simulink model "gtm_design"  (R2020b)
settings: Solver=ode3  StartTime=0.0  StopTime=20  FixedStep=Timestep  MaxStep=0.1  MinStep=0.005  RelTol=1e-5
StopFcn:
  | MWSout=grabmws(bdroot);
  | MWSout.lastrun=datestr(now);
values from neighbouring files (symbols this model uses):
  AILL = simout.surf.AILL.Data    [plot_result.m]
  AILR = simout.surf.AILR.Data    [plot_result.m]
  ELLIB = simout.surf.ELLIB.Data    [plot_result.m]
  ELLOB = simout.surf.ELLOB.Data    [plot_result.m]
  ELRIB = simout.surf.ELRIB.Data    [plot_result.m]
  ELROB = simout.surf.ELROB.Data    [plot_result.m]
  RUDL = simout.surf.RUDL.Data    [plot_result.m]
  RUDU = simout.surf.RUDU.Data    [plot_result.m]
  THROTL = simout.surf.THROTL.Data    [plot_result.m]
  THROTR = simout.surf.THROTR.Data    [plot_result.m]
undefined symbols (not defined in the file or in its folder): Aero, aftfuel, aftfuel_pos, AILLC, AILRC, alpha_deg, altitude_ft, Ax_g, Ay_g, Az_g, b, beta_deg, bias, BRAKEC, Cbar, cg_pos0, cg_shift_gear, DamageCase, DamageModels, DamageOnsetTime, ELLIBC, ELLOBC, ELRIBC, ELROBC, engl_ang, engl_pos, engr_ang, engr_pos, FLAPLIB, FLAPLIC, FLAPLOB, FLAPLOC, FLAPRIB, FLAPRIC, FLAPROB, FLAPROC, FuelUsed_Init, fwdfuel, fwdfuel_pos, GEAR, GEARC, Inertia0, Inertia_shift_gear, Ixx_model, Iyy_model, Izz_model, KTAS, LandingGear, LengON, LinearizeModeOn, NAV_altitude_m, NAV_latitude_deg, NAV_longitude_deg, NAV_Ve_mps, NAV_Vn_mps, NAV_Vu_mps, Newton, p_deg, phi_deg, POS_hi ... (+40)
libraries: simulink_need_slupdate x40, simulink x4, simulink_extras x3, UserContent_lib x1
(part 4 of 6)

== system gtm_design/GTM_T2/Actuators/Acutator Dynamics/RudderLServo ==
  In : Inport
  Constant : Constant  Value=Bias
  Gain : Gain  Gain=2*pi*freq  SaturateOnIntegerOverflow=on  OutDataTypeStr=Inherit: Same as input  ParamDataTypeStr=Inherit: Same as input
  Integrator : Integrator  InitialConditionSource=external  LimitOutput=on  UpperSaturationLimit=POS_hi  LowerSaturationLimit=POS_lo  IgnoreLimit=on
  Rate Limiter : Saturate  UpperLimit=RL  LowerLimit=-RL
  Sum : Sum  Inputs=-+|  InputSameDT=on  SaturateOnIntegerOverflow=on  OutDataTypeStr=Inherit: Same as first input
  Sum1 : Sum  Inputs=++|  InputSameDT=on  SaturateOnIntegerOverflow=on  OutDataTypeStr=Inherit: Same as first input
  Out : Outport  PortDimensions=1  VectorParamsAs1DForOutWhenUnconnected=off
  wires:
  Constant/1 -> Sum1/1
  Sum1/1 -> Integrator/2, Sum/2
  In/1 -> Sum1/2
  Rate Limiter/1 -> Integrator/1  "Ydot_lim"
  Integrator/1 -> Out/1, Sum/1  "Y"
  Sum/1 -> Gain/1  "Error"
  Gain/1 -> Rate Limiter/1  "Ydot"

== system gtm_design/GTM_T2/Actuators/Acutator Dynamics/RudderUServo ==
  In : Inport
  Constant : Constant  Value=Bias
  Gain : Gain  Gain=2*pi*freq  SaturateOnIntegerOverflow=on  OutDataTypeStr=Inherit: Same as input  ParamDataTypeStr=Inherit: Same as input
  Integrator : Integrator  InitialConditionSource=external  LimitOutput=on  UpperSaturationLimit=POS_hi  LowerSaturationLimit=POS_lo  IgnoreLimit=on
  Rate Limiter : Saturate  UpperLimit=RL  LowerLimit=-RL
  Sum : Sum  Inputs=-+|  InputSameDT=on  SaturateOnIntegerOverflow=on  OutDataTypeStr=Inherit: Same as first input
  Sum1 : Sum  Inputs=++|  InputSameDT=on  SaturateOnIntegerOverflow=on  OutDataTypeStr=Inherit: Same as first input
  Out : Outport  PortDimensions=1  VectorParamsAs1DForOutWhenUnconnected=off
  wires:
  Constant/1 -> Sum1/1
  Sum1/1 -> Integrator/2, Sum/2
  In/1 -> Sum1/2
  Rate Limiter/1 -> Integrator/1  "Ydot_lim"
  Integrator/1 -> Out/1, Sum/1  "Y"
  Sum/1 -> Gain/1  "Error"
  Gain/1 -> Rate Limiter/1  "Ydot"

== system gtm_design/GTM_T2/Actuators/Acutator Dynamics/SteeringServo ==
  In : Inport
  Constant : Constant  Value=Bias
  Gain : Gain  Gain=2*pi*freq  SaturateOnIntegerOverflow=on  OutDataTypeStr=Inherit: Same as input  ParamDataTypeStr=Inherit: Same as input
  Integrator : Integrator  InitialConditionSource=external  LimitOutput=on  UpperSaturationLimit=POS_hi  LowerSaturationLimit=POS_lo  IgnoreLimit=on
  Rate Limiter : Saturate  UpperLimit=RL  LowerLimit=-RL
  Sum : Sum  Inputs=-+|  InputSameDT=on  SaturateOnIntegerOverflow=on  OutDataTypeStr=Inherit: Same as first input
  Sum1 : Sum  Inputs=++|  InputSameDT=on  SaturateOnIntegerOverflow=on  OutDataTypeStr=Inherit: Same as first input
  Out : Outport  PortDimensions=1  VectorParamsAs1DForOutWhenUnconnected=off
  wires:
  Constant/1 -> Sum1/1
  Sum1/1 -> Integrator/2, Sum/2
  In/1 -> Sum1/2
  Rate Limiter/1 -> Integrator/1  "Ydot_lim"
  Integrator/1 -> Out/1, Sum/1  "Y"
  Sum/1 -> Gain/1  "Error"
  Gain/1 -> Rate Limiter/1  "Ydot"

== system gtm_design/GTM_T2/Actuators/DeadBand/Deadband ==
  In : Inport
  Bus Assignment : BusAssignment  AssignedSignals=ELLOB,ELLIB,ELROB,ELRIB,AILL,AILR,RUDU,RUDL,FLAPLIB,FLAPLOB,FLAPRIB,FLAPROB
  Bus Selector : BusSelector  OutputSignals=ELLOB,ELLIB,ELROB,ELRIB,AILL,AILR,RUDU,RUDL,FLAPLIB,FLAPLOB,FLAPRIB,FLAPROB
  Dead Zone : DeadZone  LowerValue=-0.3  UpperValue=0.3  SaturateOnIntegerOverflow=on
  Dead Zone1 : DeadZone  LowerValue=-0.6  UpperValue=0.6  SaturateOnIntegerOverflow=on
  Dead Zone{6,12..15} (5 alike) : DeadZone  LowerValue=-0.4  UpperValue=0.4  SaturateOnIntegerOverflow=on
  Dead Zone2 : DeadZone  LowerValue=-0.3  UpperValue=0.3  SaturateOnIntegerOverflow=on
  Dead Zone3 : DeadZone  LowerValue=-0.6  UpperValue=0.6  SaturateOnIntegerOverflow=on
  Dead Zone4 : DeadZone  LowerValue=-0.25  UpperValue=0.25  SaturateOnIntegerOverflow=on
  Dead Zone5 : DeadZone  LowerValue=-0.25  UpperValue=0.25  SaturateOnIntegerOverflow=on
  Dead Zone7 : DeadZone  LowerValue=-0.3  UpperValue=0.3  SaturateOnIntegerOverflow=on
  Out : Outport  VectorParamsAs1DForOutWhenUnconnected=off
  wires:
  Bus Selector/1 -> Dead Zone/1  "<ELLOB>"
  Bus Selector/2 -> Dead Zone1/1  "<ELLIB>"
  Bus Selector/3 -> Dead Zone2/1  "<ELROB>"
  Bus Selector/4 -> Dead Zone3/1  "<ELRIB>"
  Bus Selector/5 -> Dead Zone4/1  "<AILL>"
  Bus Selector/6 -> Dead Zone5/1  "<AILR>"
  Bus Selector/7 -> Dead Zone6/1  "<RUDU>"
  Bus Selector/8 -> Dead Zone7/1  "<RUDL>"
  Bus Selector/9 -> Dead Zone12/1  "<FLAPLIB>"
  Bus Selector/10 -> Dead Zone13/1  "<FLAPLOB>"
  Bus Selector/11 -> Dead Zone14/1  "<FLAPRIB>"
  Bus Selector/12 -> Dead Zone15/1  "<FLAPROB>"
  Dead Zone/1 -> Bus Assignment/2
  Dead Zone1/1 -> Bus Assignment/3
  Dead Zone2/1 -> Bus Assignment/4
  Dead Zone3/1 -> Bus Assignment/5
  Dead Zone4/1 -> Bus Assignment/6
  Dead Zone5/1 -> Bus Assignment/7
  Dead Zone6/1 -> Bus Assignment/8
  Dead Zone7/1 -> Bus Assignment/9
  Dead Zone12/1 -> Bus Assignment/10
  Dead Zone13/1 -> Bus Assignment/11
  Dead Zone14/1 -> Bus Assignment/12
  Dead Zone15/1 -> Bus Assignment/13
  In/1 -> Bus Assignment/1, Bus Selector/1
  Bus Assignment/1 -> Out/1

== system gtm_design/GTM_T2/Actuators/InputModification for Trimming/Invalid, Error Out ==
  Action Port : ActionPort  ActionPortLabel=default:
  Constant1 : Constant  Value=zeros(22,1)
  Constant2 : Constant  Value=0
  InvalidMode : Assertion  AssertionFailFcn="warndlg('Invalid settings for TrimMode and LinearizeMode.  Run setup.m to reset.','Warning!')"
  Out : Outport  InitialOutput=zeros(22,1)  VectorParamsAs1DForOutWhenUnconnected=off
  wires:
  Constant1/1 -> Out/1
  Constant2/1 -> InvalidMode/1

== system gtm_design/GTM_T2/Actuators/InputModification for Trimming/LinearizeMode:DetlasOnTrimBias ==
  In1 : Inport
  Action Port : ActionPort  ActionPortLabel=case [ 2 ]:
  Surface Allocation For Linearizing : Subsystem
  Out : Outport  VectorParamsAs1DForOutWhenUnconnected=off
  wires:
  Surface Allocation For Linearizing/1(O) -> Out/1
  In1/1 -> Surface Allocation For Linearizing/1(I)

== system gtm_design/GTM_T2/Actuators/InputModification for Trimming/SimMode:PassThroughWithStab ==
  Cmd : Inport
  Action Port : ActionPort  ActionPortLabel=case [ 0 ]:
  Demux7 : Demux  Outputs=[4+2+2+4+4, 1+1+2+1]
  Gain : Gain
  Gain1 : Gain
  Mux : Mux  Inputs=3
  Set with a wrench on T2/T3 : Constant  Value=bias.stabilizer
  Out : Outport  InitialOutput=zeros(22,1)  VectorParamsAs1DForOutWhenUnconnected=off
  wires:
  Cmd/1 -> Demux7/1
  Set with a wrench on T2/T3/1 -> Mux/2
  Mux/1 -> Out/1
  Demux7/1 -> Gain1/1  "Elevator(4)Aileron(2),Rudder(2),Spoliers(4),Flaps(4)"
  Demux7/2 -> Gain/1  "Gear,Brakes,Throttle(2),Steering"
  Gain1/1 -> Mux/1
  Gain/1 -> Mux/3

== system gtm_design/GTM_T2/Actuators/InputModification for Trimming/TrimMode: DriveFromTopLevel ==
  TrimBias : Inport
  Action Port : ActionPort  ActionPortLabel=case [ 1 ]:
  Bus Assignment : BusAssignment  AssignedSignals=ELLOB,ELLIB,ELROB,ELRIB,STAB,AILL,AILR,RUDU,RUDL,THROTL,THROTR,FLAPLIB,FLAPLOB,FLAPRIB,FLAPROB,GEAR,SPLLIB,SPLLOB,SPLRIB,SPLROB
  Constant1 : Constant  Value=TrimWithStab
  Demux : Demux
  Demux1 : Demux  Outputs=5
  Demux2 : Demux  Outputs=2
  Demux3 : Demux  Outputs=2
  Demux4 : Demux  Outputs=2
  Demux5 : Demux
  Demux6 : Demux
  Flaps : Constant  Value=bias.flaps
  Flaps1 : Constant  Value=bias.speedbrake
  Force Consistent Sample Time on Bus : Subsystem
  Gear : Constant  Value=bias.geardown
  InitializeBus : Subsystem
  Map : Gain  Gain=[-1;1]
  Map1 : Gain  Gain=[1;1]
  Map2 : Gain  Gain=[1;1]
  Map3 : Gain  Gain=[1;1;1;1]
  Map4 : Gain  Gain=[1;1;1;1]
  MapPitchSurf : Subsystem
  Out : Outport  InitialOutput=zeros(22,1)  VectorParamsAs1DForOutWhenUnconnected=off
  wires:
  Bus Assignment/1 -> Force Consistent Sample Time on Bus/1(In1)
  Force Consistent Sample Time on Bus/1(Out1) -> Out/1
  InitializeBus/1(O) -> Bus Assignment/1
  MapPitchSurf/1(Out) -> Demux1/1
  Demux6/4 -> Bus Assignment/21
  Demux6/3 -> Bus Assignment/20
  Demux6/2 -> Bus Assignment/19
  Demux6/1 -> Bus Assignment/18
  Map4/1 -> Demux6/1
  Flaps1/1 -> Map4/1
  Gear/1 -> Bus Assignment/17
  Map3/1 -> Demux5/1
  Demux5/4 -> Bus Assignment/16
  Demux5/3 -> Bus Assignment/15
  Demux5/2 -> Bus Assignment/14
  Demux5/1 -> Bus Assignment/13
  Flaps/1 -> Map3/1
  Map1/1 -> Demux3/1
  Demux4/2 -> Bus Assignment/12
  Demux4/1 -> Bus Assignment/11
  Map2/1 -> Demux4/1
  Demux3/2 -> Bus Assignment/10
  Demux3/1 -> Bus Assignment/9
  Demux2/2 -> Bus Assignment/8
  Demux2/1 -> Bus Assignment/7
  Map/1 -> Demux2/1
  Demux1/5 -> Bus Assignment/6
  Demux1/4 -> Bus Assignment/5
  Demux1/3 -> Bus Assignment/4
  Demux1/2 -> Bus Assignment/3
  Demux1/1 -> Bus Assignment/2
  Constant1/1 -> MapPitchSurf/1(UseStab)
  Demux/4 -> Map2/1  "Throttle"
  Demux/3 -> Map1/1  "Rudder"
  Demux/2 -> Map/1  "Aileron"
  Demux/1 -> MapPitchSurf/2(In)  "PitchSurf"
  TrimBias/1 -> Demux/1

== system gtm_design/GTM_T2/Aero/Basic Airframe/DamageEffects ==
  alpha : Inport
  beta : Inport  Port=2
  damage_case : Inport  Port=3
  Merge : Merge  InitialOutput=zeros(6,1)
  Switch Case : SwitchCase  CaseConditions={[1,2,3,4,5,6]}
  Switch Case Action Subsystem : Subsystem  TreatAsAtomicUnit=on
  Switch Case Action Subsystem2 : Subsystem  TreatAsAtomicUnit=on
  damage_case_DUP : InportShadow  Port=3
  dC6_dam : Outport  VectorParamsAs1DForOutWhenUnconnected=off
  wires:
  damage_case_DUP/1 -> Switch Case Action Subsystem/3(damage_case)
  Switch Case Action Subsystem/1(dC6_dam) -> Merge/1
  Switch Case/1 -> Switch Case Action Subsystem/Action
  damage_case/1 -> Switch Case/1
  Merge/1 -> dC6_dam/1
  beta/1 -> Switch Case Action Subsystem/2(beta)
  alpha/1 -> Switch Case Action Subsystem/1(alpha)
  Switch Case Action Subsystem2/1(Zeros) -> Merge/2
  Switch Case/2 -> Switch Case Action Subsystem2/Action

== system gtm_design/GTM_T2/Aero/Coefficent Evaluation/3D Vector Cross Product ==
  A : Inport
  B : Inport  Port=2
  Demux : Demux  Outputs=3
      settings: DisplayOption=none
  Demux1 : Demux  Outputs=3
      settings: DisplayOption=none
  Gain : Gain  Gain=-1  SaturateOnIntegerOverflow=on  OutDataTypeStr=Inherit: Same as input  ParamDataTypeStr=Inherit: Same as input
  Ground : Ground
  Mux : Mux  Inputs=9
  Product : Product  Multiplication=Matrix(*)  SaturateOnIntegerOverflow=on  OutDataTypeStr=Inherit: Same as first input
  Reshape : Reshape  OutputDimensionality=Customize  OutputDimensions=[3,3]
  AxB : Outport  VectorParamsAs1DForOutWhenUnconnected=off
  wires:
  A/1 -> Demux/1, Gain/1
  Product/1 -> AxB/1
  Ground/1 -> Mux/1, Mux/5, Mux/9
  Gain/1 -> Demux1/1
  Demux/3 -> Mux/2
  Demux1/2 -> Mux/3
  Demux1/3 -> Mux/4
  Demux/1 -> Mux/6
  Demux/2 -> Mux/7
  Demux1/1 -> Mux/8
  Mux/1 -> Reshape/1
  Reshape/1 -> Product/1
  B/1 -> Product/2

== system gtm_design/GTM_T2/Aero/Control Surfaces/Ailerons ==
  note: Basic Airframe
  note: Basic Airframe
  alpha : Inport
  beta : Inport  Port=2
  TAS : Inport  Port=3
  AC_Params : Inport  Port=4
  AILL : Inport  Port=5
  AILR : Inport  Port=6
  pqr : Inport  Port=7
  Add : Sum
  Add1 : Sum
  Basic Airframe Damage Increments : Subsystem  TreatAsAtomicUnit=on
  Basic Airframe Damage Increments1 : Subsystem  TreatAsAtomicUnit=on
  Dynamic Derviatives Damage Increments : Subsystem
  Dynamic Derviatives Damage Increments1 : Subsystem
  Gain : Gain  Gain=1/25
  Gain1 : Gain  Gain=-1
  Gain3 : Gain  Gain=1/25
  Negate Lateral1 : Gain  Gain=[1 -1 1 -1 1 -1]
  Product : Product
  Product1 : Product
  Left : Outport  VectorParamsAs1DForOutWhenUnconnected=off
  Right : Outport  Port=2  VectorParamsAs1DForOutWhenUnconnected=off
  wires:
  Dynamic Derviatives Damage Increments/1(dC6) -> Add/2
  Basic Airframe Damage Increments/1(dC6_dam) -> Add/1
  Add/1 -> Product/1
  Gain/1 -> Product/2
  Product/1 -> Left/1
  alpha/1 -> Dynamic Derviatives Damage Increments1/1(alpha), Basic Airframe Damage Increments1/1(alpha), Dynamic Derviatives Damage Increments/1(alpha), Basic Airframe Damage Increments/1(alpha)
  beta/1 -> Gain1/1, Basic Airframe Damage Increments/2(beta)
  AC_Params/1 -> Dynamic Derviatives Damage Increments1/4(AC_Params), Dynamic Derviatives Damage Increments/4(AC_Params)
  pqr/1 -> Dynamic Derviatives Damage Increments1/3(pqr), Dynamic Derviatives Damage Increments/3(pqr)
  AILL/1 -> Gain/1
  Add1/1 -> Product1/1
  Basic Airframe Damage Increments1/1(dC6_dam) -> Add1/1
  Dynamic Derviatives Damage Increments1/1(dC6) -> Add1/2
  Gain1/1 -> Basic Airframe Damage Increments1/2(beta)
  AILR/1 -> Gain3/1
  Gain3/1 -> Product1/2
  Product1/1 -> Negate Lateral1/1
  Negate Lateral1/1 -> Right/1
  TAS/1 -> Dynamic Derviatives Damage Increments1/2(TAS), Dynamic Derviatives Damage Increments/2(TAS)

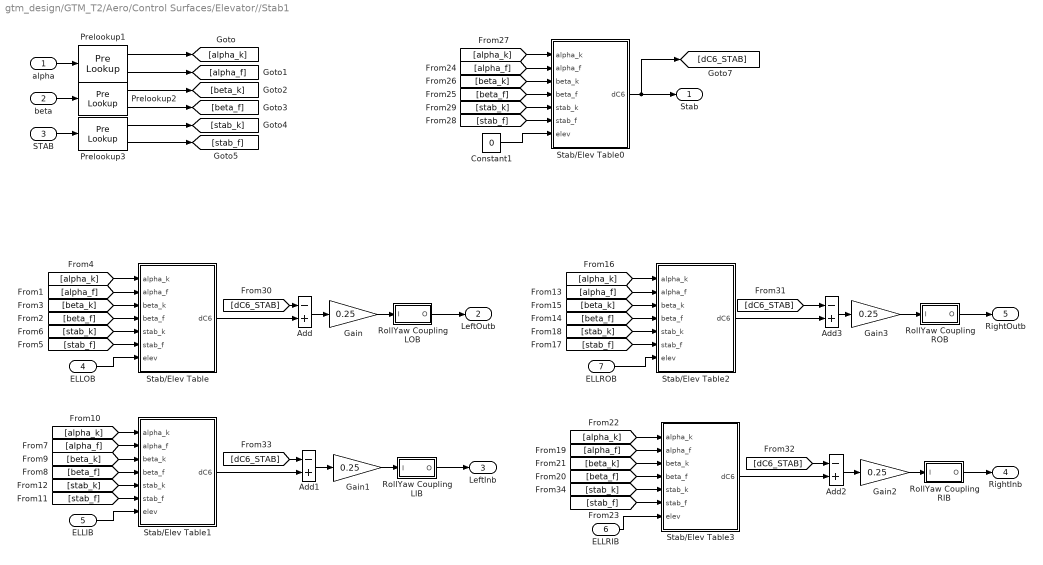
== system gtm_design/GTM_T2/Aero/Control Surfaces/Elevator//Stab1 ==
  alpha : Inport
  beta : Inport  Port=2
  STAB : Inport  Port=3
  ELLOB : Inport  Port=4
  ELLIB : Inport  Port=5
  ELLRIB : Inport  Port=6
  ELLROB : Inport  Port=7
  Add{,1..3} (4 alike) : Sum  Inputs=-+
  Constant1 : Constant  Value=0
  Gain{,1..3} (4 alike) : Gain  Gain=0.25
  Prelookup1 : PreLookup  BreakpointsData=Aero.dC3_ele.alpha  IndexSearchMethod=Linear search  BeginIndexSearchUsingPreviousIndexResult=on  ExtrapMethod=Linear
  Prelookup2 : PreLookup  BreakpointsData=Aero.dC3_ele.beta  IndexSearchMethod=Linear search  BeginIndexSearchUsingPreviousIndexResult=on  ExtrapMethod=Linear
  Prelookup3 : PreLookup  BreakpointsData=Aero.dC3_ele.stab  IndexSearchMethod=Linear search  BeginIndexSearchUsingPreviousIndexResult=on  ExtrapMethod=Linear
  RollYaw Coupling LIB : Subsystem  mask{arm=-0.03}
      mask prompts: arm "Moment arm (nd)"
      mask help:
      | Approximates roll/yaw coupling of split longitudinal surface
      | deflections (spoilers, elevators, flaps) where the base aero data only
      | has CX, CZ, and Cm. Input should be a 6 element vector of the aero
      | coefficients [CZ CY CZ Cl Cm Cn].
      |
      | Cl = Cl_input + arm*CZ_input
      | Cn = Cn_input + arm*CX_input
      mask init:
      | Kc = eye(6);
      | 
      | Kc(4,3) = arm; % Cl = Cl + arm*CZ
      | Kc(6,1) = -arm; % Cn = Cn - arm*CX
  RollYaw Coupling LOB : Subsystem  mask{arm=-0.07}
      mask prompts: arm "Moment arm (nd)"
      mask help:
      | Approximates roll/yaw coupling of split longitudinal surface
      | deflections (spoilers, elevators, flaps) where the base aero data only
      | has CX, CZ, and Cm. Input should be a 6 element vector of the aero
      | coefficients [CZ CY CZ Cl Cm Cn].
      |
      | Cl = Cl_input + arm*CZ_input
      | Cn = Cn_input + arm*CX_input
      mask init:
      | Kc = eye(6);
      | 
      | Kc(4,3) = arm; % Cl = Cl + arm*CZ
      | Kc(6,1) = -arm; % Cn = Cn - arm*CX
  RollYaw Coupling RIB : Subsystem  mask{arm=0.03}
      mask prompts: arm "Moment arm (nd)"
      mask help:
      | Approximates roll/yaw coupling of split longitudinal surface
      | deflections (spoilers, elevators, flaps) where the base aero data only
      | has CX, CZ, and Cm. Input should be a 6 element vector of the aero
      | coefficients [CZ CY CZ Cl Cm Cn].
      |
      | Cl = Cl_input + arm*CZ_input
      | Cn = Cn_input + arm*CX_input
      mask init:
      | Kc = eye(6);
      | 
      | Kc(4,3) = arm; % Cl = Cl + arm*CZ
      | Kc(6,1) = -arm; % Cn = Cn - arm*CX
  RollYaw Coupling ROB : Subsystem  mask{arm=0.07}
      mask prompts: arm "Moment arm (nd)"
      mask help:
      | Approximates roll/yaw coupling of split longitudinal surface
      | deflections (spoilers, elevators, flaps) where the base aero data only
      | has CX, CZ, and Cm. Input should be a 6 element vector of the aero
      | coefficients [CZ CY CZ Cl Cm Cn].
      |
      | Cl = Cl_input + arm*CZ_input
      | Cn = Cn_input + arm*CX_input
      mask init:
      | Kc = eye(6);
      | 
      | Kc(4,3) = arm; % Cl = Cl + arm*CZ
      | Kc(6,1) = -arm; % Cn = Cn - arm*CX
  Stab/Elev Table : Subsystem
  Stab/Elev Table0 : Subsystem
  Stab/Elev Table1 : Subsystem
  Stab/Elev Table2 : Subsystem
  Stab/Elev Table3 : Subsystem
  Stab : Outport  VectorParamsAs1DForOutWhenUnconnected=off
  LeftOutb : Outport  Port=2  VectorParamsAs1DForOutWhenUnconnected=off
  LeftInb : Outport  Port=3  VectorParamsAs1DForOutWhenUnconnected=off
  RightInb : Outport  Port=4  VectorParamsAs1DForOutWhenUnconnected=off
  RightOutb : Outport  Port=5  VectorParamsAs1DForOutWhenUnconnected=off
  wires:
  RollYaw Coupling RIB/1(O) -> RightInb/1
  RollYaw Coupling ROB/1(O) -> RightOutb/1
  RollYaw Coupling LIB/1(O) -> LeftInb/1
  RollYaw Coupling LOB/1(O) -> LeftOutb/1
  Stab/Elev Table0/1(dC6) -> [dC6_STAB], Stab/1
  [dC6_STAB] -> Add1/1
  Stab/Elev Table3/1(dC6) -> Add2/2
  [dC6_STAB] -> Add2/1
  [dC6_STAB] -> Add3/1
  Stab/Elev Table2/1(dC6) -> Add3/2
  Stab/Elev Table1/1(dC6) -> Add1/2
  Constant1/1 -> Stab/Elev Table0/7(elev)
  [stab_f] -> Stab/Elev Table0/6(stab_f)
  [stab_k] -> Stab/Elev Table0/5(stab_k)
  [beta_f] -> Stab/Elev Table0/4(beta_f)
  [beta_k] -> Stab/Elev Table0/3(beta_k)
  [alpha_f] -> Stab/Elev Table0/2(alpha_f)
  [alpha_k] -> Stab/Elev Table0/1(alpha_k)
  [dC6_STAB] -> Add/1
  Stab/Elev Table/1(dC6) -> Add/2
  ELLRIB/1 -> Stab/Elev Table3/7(elev)
  [stab_f] -> Stab/Elev Table3/6(stab_f)
  [stab_k] -> Stab/Elev Table3/5(stab_k)
  [beta_f] -> Stab/Elev Table3/4(beta_f)
  [beta_k] -> Stab/Elev Table3/3(beta_k)
  [alpha_f] -> Stab/Elev Table3/2(alpha_f)
  [alpha_k] -> Stab/Elev Table3/1(alpha_k)
  ELLROB/1 -> Stab/Elev Table2/7(elev)
  [stab_f] -> Stab/Elev Table2/6(stab_f)
  [stab_k] -> Stab/Elev Table2/5(stab_k)
  [beta_f] -> Stab/Elev Table2/4(beta_f)
  [beta_k] -> Stab/Elev Table2/3(beta_k)
  [alpha_f] -> Stab/Elev Table2/2(alpha_f)
  [alpha_k] -> Stab/Elev Table2/1(alpha_k)
  ELLIB/1 -> Stab/Elev Table1/7(elev)
  [stab_f] -> Stab/Elev Table1/6(stab_f)
  [stab_k] -> Stab/Elev Table1/5(stab_k)
  [beta_f] -> Stab/Elev Table1/4(beta_f)
  [beta_k] -> Stab/Elev Table1/3(beta_k)
  [alpha_f] -> Stab/Elev Table1/2(alpha_f)
  [alpha_k] -> Stab/Elev Table1/1(alpha_k)
  ELLOB/1 -> Stab/Elev Table/7(elev)
  [stab_f] -> Stab/Elev Table/6(stab_f)
  [stab_k] -> Stab/Elev Table/5(stab_k)
  [beta_f] -> Stab/Elev Table/4(beta_f)
  [beta_k] -> Stab/Elev Table/3(beta_k)
  [alpha_f] -> Stab/Elev Table/2(alpha_f)
  [alpha_k] -> Stab/Elev Table/1(alpha_k)
  Add3/1 -> Gain3/1
  Add2/1 -> Gain2/1
  Add1/1 -> Gain1/1
  Add/1 -> Gain/1
  Gain3/1 -> RollYaw Coupling ROB/1(I)
  Gain2/1 -> RollYaw Coupling RIB/1(I)
  Gain1/1 -> RollYaw Coupling LIB/1(I)
  Gain/1 -> RollYaw Coupling LOB/1(I)
  Prelookup3/2 -> [stab_f]
  Prelookup3/1 -> [stab_k]
  Prelookup2/2 -> [beta_f]
  Prelookup2/1 -> [beta_k]
  Prelookup1/2 -> [alpha_f]
  Prelookup1/1 -> [alpha_k]
  STAB/1 -> Prelookup3/1
  beta/1 -> Prelookup2/1
  alpha/1 -> Prelookup1/1

== system gtm_design/GTM_T2/Aero/Control Surfaces/Flaps ==
  alpha : Inport
  FLAPLOB : Inport  Port=2
  FLAPLIB : Inport  Port=3
  FLAPRIB : Inport  Port=4
  FLAPROB : Inport  Port=5
  Gain : Gain  Gain=Aero.flaps.flaplob
  Gain1 : Gain  Gain=Aero.flaps.flaplib
  Gain2 : Gain  Gain=Aero.flaps.flaprib
  Gain3 : Gain  Gain=Aero.flaps.flaprob
  Terminator : Terminator
  LeftOutb : Outport  VectorParamsAs1DForOutWhenUnconnected=off
  LeftInb : Outport  Port=2  VectorParamsAs1DForOutWhenUnconnected=off
  RightInb : Outport  Port=3  VectorParamsAs1DForOutWhenUnconnected=off
  RightOutb : Outport  Port=4  VectorParamsAs1DForOutWhenUnconnected=off
  wires:
  Gain3/1 -> RightOutb/1
  Gain2/1 -> RightInb/1
  Gain1/1 -> LeftInb/1
  Gain/1 -> LeftOutb/1
  FLAPROB/1 -> Gain3/1
  FLAPRIB/1 -> Gain2/1
  FLAPLIB/1 -> Gain1/1
  FLAPLOB/1 -> Gain/1
  alpha/1 -> Terminator/1

== system gtm_design/GTM_T2/Aero/Control Surfaces/Gear ==
  alpha : Inport
  gear : Inport  Port=2
  Assignment to Longitudinal : Assignment  IndexMode=Zero-based  IndexOptions=Index vector (dialog)  Indices=[0 2 4]  OutputSizes=[1 1]
  Compare To Zero : simulink/Logic and Bit Operations/Compare To Zero  relop=~=  OutDataTypeStr=uint8  ZeroCross=off
  Constant : Constant  Value=zeros(6,1)
  Constant2 : Constant  Value=[0:2]  OutDataTypeStr=uint32
  Data Type Conversion2 : DataTypeConversion  OutDataTypeStr=uint32
  PreLookup Index Search1 : simulink_need_slupdate/PreLookup Index Search  bpData=Aero.dC3_lgr.alpha  searchMode=Binary Search  cacheBpFlag=on  outputFlag=off  IndexDataType=uint32  extrapMode=Linear Extrapolation  rangeErrorMode=None
      settings: SourceProductBaseCode=SL
  TableLookup : simulink_need_slupdate/Interpolation (n-D) using PreLookup  numDimsPopupSelect=3  explicitNumDims=2  table=Aero.dC3_lgr.data  interpMethod=Linear  extrapMethod=Linear  rangeErrorMode=None  NumSelectionDims=2
      settings: SourceProductBaseCode=SL
  LandingGear : Outport  VectorParamsAs1DForOutWhenUnconnected=off
  wires:
  gear/1 -> Compare To Zero/1
  Compare To Zero/1 -> Data Type Conversion2/1
  alpha/1 -> PreLookup Index Search1/1
  PreLookup Index Search1/1 -> TableLookup/1
  Constant2/1 -> TableLookup/3
  TableLookup/1 -> Assignment to Longitudinal/2
  Constant/1 -> Assignment to Longitudinal/1
  Assignment to Longitudinal/1 -> LandingGear/1
  Data Type Conversion2/1 -> TableLookup/2

== system gtm_design/GTM_T2/Aero/Control Surfaces/Implement Damage Models ==
  SurfVec : Inport
  damagecase : Inport  Port=2
  Implement Damage Models : MATLAB Function  TreatAsAtomicUnit=on
  Reshape : Reshape
  dC6 : Outport  VectorParamsAs1DForOutWhenUnconnected=off
  wires:
  Reshape/1 -> dC6/1
  damagecase/1 -> Implement Damage Models/2(DamageCase)
  Implement Damage Models/1(dC6) -> Reshape/1
  SurfVec/1 -> Implement Damage Models/1(SurfVec)

== system gtm_design/GTM_T2/Aero/Control Surfaces/Rudder ==
  alpha : Inport
  beta : Inport  Port=2
  RUDU : Inport  Port=3
  RUDL : Inport  Port=4
  Gains : Subsystem  mask{gains=[0.5  0.5  0.5  0.67  0.67  0.5]}
      mask prompts: gains "Mask Parameter 1:"
      mask help: Gains for each aerodynamic coefficient.
      mask Display: disp(['[' num2str(gains) ']'])
  Gains1 : Subsystem  mask{gains=[0.5  0.5  0.5  0.33  0.33  0.5]}
      mask prompts: gains "Mask Parameter 1:"
      mask help: Gains for each aerodynamic coefficient.
      mask Display: disp(['[' num2str(gains) ']'])
  Lower Rudder : Subsystem
  Upper Rudder : Subsystem
  Upper : Outport  VectorParamsAs1DForOutWhenUnconnected=off
  Lower : Outport  Port=2  VectorParamsAs1DForOutWhenUnconnected=off
  wires:
  RUDL/1 -> Lower Rudder/3(rud)
  Gains1/1(dC6) -> Lower/1
  RUDU/1 -> Upper Rudder/3(rud)
  beta/1 -> Lower Rudder/2(beta), Upper Rudder/2(beta)
  Gains/1(dC6) -> Upper/1
  alpha/1 -> Lower Rudder/1(alpha), Upper Rudder/1(alpha)
  Upper Rudder/1(dC6) -> Gains/1(dC6_in)
  Lower Rudder/1(dC6) -> Gains1/1(dC6_in)

== system gtm_design/GTM_T2/Aero/Control Surfaces/Spoilers ==
  alpha : Inport
  beta : Inport  Port=2
  SPLLIB : Inport  Port=3
  SPLRIB : Inport  Port=4
  SPLLOB : Inport  Port=5
  SPLROB : Inport  Port=6
  Gains1 : Subsystem  mask{gains=|}
      mask gains=|
      | [0.45	0.45	0.45	0.26	0.45	0.26
      | ]
      mask prompts: gains "Mask Parameter 1:"
      mask help: Gains for each aerodynamic coefficient.
      mask Display: disp(['[' num2str(gains) ']'])
  Gains2 : Subsystem  mask{gains=|}
      mask gains=|
      | [0.45	0.45	0.45	0.26	0.45	0.26
      | ]
      mask prompts: gains "Mask Parameter 1:"
      mask help: Gains for each aerodynamic coefficient.
      mask Display: disp(['[' num2str(gains) ']'])
  Gains3 : Subsystem  mask{gains=|}
      mask gains=|
      | [0.55	0.55	0.55	0.74	0.55	0.74
      | ]
      mask prompts: gains "Mask Parameter 1:"
      mask help: Gains for each aerodynamic coefficient.
      mask Display: disp(['[' num2str(gains) ']'])
  Gains4 : Subsystem  mask{gains=|}
      mask gains=|
      | [0.55	0.55	0.55	0.74	0.55	0.74
      | ]
      mask prompts: gains "Mask Parameter 1:"
      mask help: Gains for each aerodynamic coefficient.
      mask Display: disp(['[' num2str(gains) ']'])
  InboardSpoilers : Subsystem
  OutboardSpoilers : Subsystem
  LeftInb : Outport  VectorParamsAs1DForOutWhenUnconnected=off
  LeftOutb : Outport  Port=2  VectorParamsAs1DForOutWhenUnconnected=off
  RightInb : Outport  Port=3  VectorParamsAs1DForOutWhenUnconnected=off
  RightOutb : Outport  Port=4  VectorParamsAs1DForOutWhenUnconnected=off
  wires:
  Gains4/1(dC6) -> RightOutb/1
  OutboardSpoilers/2(Right) -> Gains4/1(dC6_in)
  Gains1/1(dC6) -> RightInb/1
  InboardSpoilers/2(Right) -> Gains1/1(dC6_in)
  SPLROB/1 -> OutboardSpoilers/4(SPLRIB)
  SPLLOB/1 -> OutboardSpoilers/3(SPLLIB)
  Gains3/1(dC6) -> LeftOutb/1
  SPLRIB/1 -> InboardSpoilers/4(SPLRIB)
  SPLLIB/1 -> InboardSpoilers/3(SPLLIB)
  Gains2/1(dC6) -> LeftInb/1
  beta/1 -> OutboardSpoilers/2(beta), InboardSpoilers/2(beta)
  alpha/1 -> OutboardSpoilers/1(alpha), InboardSpoilers/1(alpha)
  OutboardSpoilers/1(Left) -> Gains3/1(dC6_in)
  InboardSpoilers/1(Left) -> Gains2/1(dC6_in)

== system gtm_design/GTM_T2/Aero/Dynamic Derviatives/Forced Oscillation with Damage Increments ==
  alpha : Inport
  TAS : Inport  Port=2
  pqr : Inport  Port=3
  AC_Params : Inport  Port=4
  DamageCase : Inport  Port=5
  Action Port : ActionPort  ActionPortLabel=case [ 1 2 3 4 5 6 ]:
  Add : Sum  Inputs=+++
  Add1 : Sum
  Assignment to CY : Assignment  IndexMode=Zero-based  IndexOptions=Index vector (dialog)  Indices=1  OutputSizes=[1 1]
  Constant4 : Constant  Value=zeros(6,1)
  Damage Effects-Increments : Subsystem
  Damage Effects-Scaling : Subsystem
  Forced Oscillation : Subsystem
  Normalize : Subsystem
  Product1 : Product  RndMeth=Zero
  Product2 : Product  RndMeth=Zero
  Product3 : Product  RndMeth=Zero
  dC6 : Outport  VectorParamsAs1DForOutWhenUnconnected=off
  wires:
  Assignment to CY/1 -> Add1/1
  Add/1 -> Add1/2
  Product2/1 -> Add/1
  Product1/1 -> Add/2
  Product3/1 -> Add/3
  Forced Oscillation/3(dC6_r) -> Product3/2
  Forced Oscillation/2(dC6_q) -> Product1/2
  Forced Oscillation/1(dC6_p) -> Product2/2
  Normalize/1(pqrhat) -> Damage Effects-Increments/2(pqr), Forced Oscillation/2(pqr)
  AC_Params/1 -> Normalize/3(AC_Params)
  TAS/1 -> Normalize/2(TAS)
  pqr/1 -> Normalize/1(pqr)
  Add1/1 -> dC6/1
  Constant4/1 -> Assignment to CY/1
  Damage Effects-Increments/1(Increment) -> Assignment to CY/2
  Damage Effects-Scaling/3(Scaling_p) -> Product2/1
  Damage Effects-Scaling/2(Scaling_q) -> Product1/1
  Damage Effects-Scaling/1(Scaling_r) -> Product3/1
  DamageCase/1 -> Damage Effects-Increments/3(DamageCase), Damage Effects-Scaling/2(DamageCase)
  alpha/1 -> Damage Effects-Increments/1(alpha), Damage Effects-Scaling/1(alpha), Forced Oscillation/1(alpha)

== system gtm_design/GTM_T2/Aero/Dynamic Derviatives/Rotary Blended UnDamaged Case ==
  alpha : Inport
  beta : Inport  Port=2
  TAS : Inport  Port=3
  pqr : Inport  Port=4
  AC_Params : Inport  Port=5
  Action Port : ActionPort  ActionPortLabel=default:
  Add : Sum  Inputs=++++
  Blending Function : MATLAB Function  TreatAsAtomicUnit=on
  Bus Selector2 : BusSelector  OutputSignals=B,Cbar
  Forced Oscillation : Subsystem
  Rotary Balance : Subsystem
  Saturation : Saturate
  Saturation1 : Saturate  UpperLimit=10000  LowerLimit=1
  dC6 : Outport  VectorParamsAs1DForOutWhenUnconnected=off
  wires:
  Forced Oscillation/3(dC6_r) -> Add/4
  Forced Oscillation/2(dC6_q) -> Add/3
  Forced Oscillation/1(dC6_p) -> Add/2
  Rotary Balance/1(dC6) -> Add/1
  Add/1 -> dC6/1
  Bus Selector2/2 -> Blending Function/6(Cbar)  "<Cbar>"
  pqr/1 -> Blending Function/4(pqr)
  Saturation1/1 -> Blending Function/3(tas)
  Saturation/1 -> Rotary Balance/3(w)
  [alpha] -> Forced Oscillation/1(alpha)
  [beta] -> Rotary Balance/2(beta)
  [alpha] -> Rotary Balance/1(alpha)
  [beta] -> Blending Function/2(beta)
  beta/1 -> [beta]
  alpha/1 -> [alpha]
  [alpha] -> Blending Function/1(alpha)
  AC_Params/1 -> Bus Selector2/1
  TAS/1 -> Saturation1/1
  Bus Selector2/1 -> Blending Function/5(B)  "<B>"
  Blending Function/2(pqr_osc) -> Forced Oscillation/2(pqr)
  Blending Function/1(omega) -> Saturation/1

== system gtm_design/GTM_T2/AuxiliaryVariables/Atmos76/Atmos List ==
  I : Inport
  BusCreator : BusCreator  Inputs=7
  Demux2 : Demux  Outputs=6
      settings: DisplayOption=none
  Divide : Product  Inputs=*/
  Standard Temp. K : Constant  Value=288.15
  O : Outport  VectorParamsAs1DForOutWhenUnconnected=off
  wires:
  Divide/1 -> BusCreator/7  "tratio"
  Standard Temp. K/1 -> Divide/2
  BusCreator/1 -> O/1
  I/1 -> Demux2/1
  Demux2/1 -> BusCreator/1  "rho"
  Demux2/2 -> BusCreator/2  "pressure"
  Demux2/3 -> Divide/1, BusCreator/3  "temperature"
  Demux2/4 -> BusCreator/4  "cs"
  Demux2/5 -> BusCreator/5  "pratio"
  Demux2/6 -> BusCreator/6  "sqrsig"

== system gtm_design/GTM_T2/AuxiliaryVariables/WindShear and Xform/WindShear ==
  note: ShearFactor = ln(h/.15) / ln(h/20), as per MIL-Spec: MIL-F-8785C
  In : Inport
  Constant2 : Constant  Value=log(20/.15);
  Divide : Product  Inputs=*/
  Gain : Gain  Gain=1/.15; %MILSpec constant
  Gain2 : Gain  Gain=1/1.8; % Scale to get unity gain@1000ft (instead of 20 ft)
  Math Function : Math  Operator=log  SignedPower=on  SaturateOnIntegerOverflow=on
  Saturation : Saturate  UpperLimit=1000  LowerLimit=1
  Out : Outport  VectorParamsAs1DForOutWhenUnconnected=off
  wires:
  Gain2/1 -> Out/1
  Saturation/1 -> Gain/1
  Divide/1 -> Gain2/1
  Constant2/1 -> Divide/2
  Math Function/1 -> Divide/1
  In/1 -> Saturation/1
  Gain/1 -> Math Function/1

== system gtm_design/GTM_T2/EOM/Aircraft 6DOF/3D Vector Cross Product ==
  A : Inport
  B : Inport  Port=2
  Demux : Demux  Outputs=3
      settings: DisplayOption=none
  Demux1 : Demux  Outputs=3
      settings: DisplayOption=none
  Gain : Gain  Gain=-1  SaturateOnIntegerOverflow=on  OutDataTypeStr=Inherit: Same as input  ParamDataTypeStr=Inherit: Same as input
  Ground : Ground
  Mux : Mux  Inputs=9
  Product : Product  Multiplication=Matrix(*)  SaturateOnIntegerOverflow=on  OutDataTypeStr=Inherit: Same as first input
  Reshape : Reshape  OutputDimensionality=Customize  OutputDimensions=[3,3]
  AxB : Outport  VectorParamsAs1DForOutWhenUnconnected=off
  wires:
  A/1 -> Demux/1, Gain/1
  Product/1 -> AxB/1
  Ground/1 -> Mux/1, Mux/5, Mux/9
  Gain/1 -> Demux1/1
  Demux/3 -> Mux/2
  Demux1/2 -> Mux/3
  Demux1/3 -> Mux/4
  Demux/1 -> Mux/6
  Demux/2 -> Mux/7
  Demux1/1 -> Mux/8
  Mux/1 -> Reshape/1
  Reshape/1 -> Product/1
  B/1 -> Product/2

== system gtm_design/GTM_T2/EOM/Aircraft 6DOF/3D Vector Cross Product1 ==
  A : Inport
  B : Inport  Port=2
  Demux : Demux  Outputs=3
      settings: DisplayOption=none
  Demux1 : Demux  Outputs=3
      settings: DisplayOption=none
  Gain : Gain  Gain=-1  SaturateOnIntegerOverflow=on  OutDataTypeStr=Inherit: Same as input  ParamDataTypeStr=Inherit: Same as input
  Ground : Ground
  Mux : Mux  Inputs=9
  Product : Product  Multiplication=Matrix(*)  SaturateOnIntegerOverflow=on  OutDataTypeStr=Inherit: Same as first input
  Reshape : Reshape  OutputDimensionality=Customize  OutputDimensions=[3,3]
  AxB : Outport  VectorParamsAs1DForOutWhenUnconnected=off
  wires:
  A/1 -> Demux/1, Gain/1
  Product/1 -> AxB/1
  Ground/1 -> Mux/1, Mux/5, Mux/9
  Gain/1 -> Demux1/1
  Demux/3 -> Mux/2
  Demux1/2 -> Mux/3
  Demux1/3 -> Mux/4
  Demux/1 -> Mux/6
  Demux/2 -> Mux/7
  Demux1/1 -> Mux/8
  Mux/1 -> Reshape/1
  Reshape/1 -> Product/1
  B/1 -> Product/2

== system gtm_design/GTM_T2/EOM/Aircraft 6DOF/Euler to DCM ==
  "Euler " : Inport
  Fcn : Fcn  Expr=u(4)*u(2)*u(6)+u(3)*u(1)
  Fcn1 : Fcn  Expr=u(3)*u(5)
  Fcn2 : Fcn  Expr=u(3)*u(2)*u(1)+u(6)*u(4)
  Fcn3 : Fcn  Expr=u(3)*u(2)*u(4)-u(6)*u(1)
  Fcn4 : Fcn  Expr=-u(2)
  Fcn5 : Fcn  Expr=u(5)*u(1)
  Fcn6 : Fcn  Expr=u(1)*u(2)*u(6)-u(3)*u(4)
  Fcn7 : Fcn  Expr=u(5)*u(6)
  Fcn8 : Fcn  Expr=u(5)*u(4)
  Mux : Mux  Inputs=2
  Mux1 : Mux  Inputs=9
  Reshape : Reshape  OutputDimensionality=Customize  OutputDimensions=[3,3]
  Trigonometric Function : Trigonometry
  Trigonometric Function1 : Trigonometry  Operator=cos
  DCM : Outport  VectorParamsAs1DForOutWhenUnconnected=off
  wires:
  "Euler "/1 -> Trigonometric Function1/1, Trigonometric Function/1
  Trigonometric Function/1 -> Mux/1
  Trigonometric Function1/1 -> Mux/2
  Mux/1 -> Fcn/1, Fcn7/1, Fcn6/1, Fcn1/1, Fcn2/1, Fcn4/1, Fcn8/1, Fcn5/1, Fcn3/1
  Mux1/1 -> Reshape/1
  Fcn7/1 -> Mux1/1
  Fcn6/1 -> Mux1/2
  Fcn/1 -> Mux1/3
  Fcn1/1 -> Mux1/4
  Fcn2/1 -> Mux1/5
  Fcn3/1 -> Mux1/6
  Fcn4/1 -> Mux1/7
  Fcn5/1 -> Mux1/8
  Fcn8/1 -> Mux1/9
  Reshape/1 -> DCM/1

== system gtm_design/GTM_T2/EOM/Aircraft 6DOF/Vlocal to LatLon ==
  I : Inport
  Constant1 : Constant  Value=-1
  "EarthRadius " : Constant  Value=Re
  Math Function1 : Math  Operator=reciprocal  SignedPower=on  SaturateOnIntegerOverflow=on
  Mux : Mux  Inputs=3
  Product : Product  Inputs=*/  RndMeth=Zero
  Selector : Selector  InputPortWidth=3  IndexOptions=Index vector (dialog)  Indices=3  OutputSizes=1
  Selector1 : Selector  InputPortWidth=3  IndexOptions=Index vector (dialog)  Indices=1  OutputSizes=1
  Sum2 : Sum  Inputs=|++
  Trigonometric Function : Trigonometry  Operator=cos
  O : Outport  VectorParamsAs1DForOutWhenUnconnected=off
  wires:
  "EarthRadius "/1 -> Sum2/2
  Sum2/1 -> Math Function1/1
  Trigonometric Function/1 -> Product/2
  Math Function1/1 -> Product/1, Mux/1
  Product/1 -> Mux/2
  Constant1/1 -> Mux/3
  Selector/1 -> Sum2/1
  I/1 -> Selector/1, Selector1/1
  Mux/1 -> O/1
  Selector1/1 -> Trigonometric Function/1

== system gtm_design/GTM_T2/EOM/Anti Windup/Subsystem1 ==
  I : Inport
  Constant1 : Constant  Value=2*pi
  Constant2 : Constant  Value=2*pi
  Constant3 : Constant  Value=2*pi
  Math Function1 : Math  Operator=rem  SignedPower=on  SaturateOnIntegerOverflow=on
  Sum : Sum  Inputs=|-+  SaturateOnIntegerOverflow=on
  Sum1 : Sum  Inputs=++|  SaturateOnIntegerOverflow=on
  Switch : Switch  Criteria=u2 > Threshold  Threshold=pi  SaturateOnIntegerOverflow=on
  Switch1 : Switch  SaturateOnIntegerOverflow=on
  Switch2 : Switch  Threshold=-pi  SaturateOnIntegerOverflow=on
  O : Outport  VectorParamsAs1DForOutWhenUnconnected=off
  wires:
  Switch1/1 -> O/1
  Switch/1 -> Switch1/1
  Switch2/1 -> Switch1/3
  Sum1/1 -> Switch2/3
  Constant3/1 -> Sum1/2
  Sum/1 -> Switch/1
  Constant2/1 -> Sum/1
  Math Function1/1 -> Switch1/2, Sum1/1, Switch2/2, Switch2/1, Switch/3, Sum/2, Switch/2
  I/1 -> Math Function1/1
  Constant1/1 -> Math Function1/2

== system gtm_design/GTM_T2/EOM/Anti Windup/Subsystem3 ==
  I : Inport
  Constant1 : Constant  Value=2*pi
  Constant2 : Constant  Value=2*pi
  Constant3 : Constant  Value=2*pi
  Math Function1 : Math  Operator=rem  SignedPower=on  SaturateOnIntegerOverflow=on
  Sum : Sum  Inputs=|-+  SaturateOnIntegerOverflow=on
  Sum1 : Sum  Inputs=++|  SaturateOnIntegerOverflow=on
  Switch : Switch  Criteria=u2 > Threshold  Threshold=pi  SaturateOnIntegerOverflow=on
  Switch1 : Switch  SaturateOnIntegerOverflow=on
  Switch2 : Switch  Threshold=-pi  SaturateOnIntegerOverflow=on
  O : Outport  VectorParamsAs1DForOutWhenUnconnected=off
  wires:
  Switch1/1 -> O/1
  Switch/1 -> Switch1/1
  Switch2/1 -> Switch1/3
  Sum1/1 -> Switch2/3
  Constant3/1 -> Sum1/2
  Sum/1 -> Switch/1
  Constant2/1 -> Sum/1
  Math Function1/1 -> Switch1/2, Sum1/1, Switch2/2, Switch2/1, Switch/3, Sum/2, Switch/2
  I/1 -> Math Function1/1
  Constant1/1 -> Math Function1/2

== system gtm_design/GTM_T2/EOM/Anti Windup/Subsystem4 ==
  I : Inport
  Constant1 : Constant  Value=2*pi
  Math Function1 : Math  Operator=rem  SignedPower=on  SaturateOnIntegerOverflow=on
  Math Function2 : Math  Operator=rem  SignedPower=on  SaturateOnIntegerOverflow=on
  Sum2 : Sum  Inputs=|++  SaturateOnIntegerOverflow=on
  O : Outport  VectorParamsAs1DForOutWhenUnconnected=off
  wires:
  Constant1/1 -> Math Function1/2, Math Function2/2, Sum2/2
  I/1 -> Math Function1/1
  Sum2/1 -> Math Function2/1
  Math Function1/1 -> Sum2/1
  Math Function2/1 -> O/1

== system gtm_design/GTM_T2/Engines/CG torque/3D Vector Cross Product ==
  A : Inport
  B : Inport  Port=2
  Demux : Demux  Outputs=3
      settings: DisplayOption=none
  Demux1 : Demux  Outputs=3
      settings: DisplayOption=none
  Gain : Gain  Gain=-1  SaturateOnIntegerOverflow=on  OutDataTypeStr=Inherit: Same as input  ParamDataTypeStr=Inherit: Same as input
  Ground : Ground
  Mux : Mux  Inputs=9
  Product : Product  Multiplication=Matrix(*)  SaturateOnIntegerOverflow=on  OutDataTypeStr=Inherit: Same as first input
  Reshape : Reshape  OutputDimensionality=Customize  OutputDimensions=[3,3]
  AxB : Outport  VectorParamsAs1DForOutWhenUnconnected=off
  wires:
  A/1 -> Demux/1, Gain/1
  Product/1 -> AxB/1
  Ground/1 -> Mux/1, Mux/5, Mux/9
  Gain/1 -> Demux1/1
  Demux/3 -> Mux/2
  Demux1/2 -> Mux/3
  Demux1/3 -> Mux/4
  Demux/1 -> Mux/6
  Demux/2 -> Mux/7
  Demux1/1 -> Mux/8
  Mux/1 -> Reshape/1
  Reshape/1 -> Product/1
  B/1 -> Product/2

== system gtm_design/GTM_T2/Engines/CG torque/3D Vector Cross Product1 ==
  A : Inport
  B : Inport  Port=2
  Demux : Demux  Outputs=3
      settings: DisplayOption=none
  Demux1 : Demux  Outputs=3
      settings: DisplayOption=none
  Gain : Gain  Gain=-1  SaturateOnIntegerOverflow=on  OutDataTypeStr=Inherit: Same as input  ParamDataTypeStr=Inherit: Same as input
  Ground : Ground
  Mux : Mux  Inputs=9
  Product : Product  Multiplication=Matrix(*)  SaturateOnIntegerOverflow=on  OutDataTypeStr=Inherit: Same as first input
  Reshape : Reshape  OutputDimensionality=Customize  OutputDimensions=[3,3]
  AxB : Outport  VectorParamsAs1DForOutWhenUnconnected=off
  wires:
  A/1 -> Demux/1, Gain/1
  Product/1 -> AxB/1
  Ground/1 -> Mux/1, Mux/5, Mux/9
  Gain/1 -> Demux1/1
  Demux/3 -> Mux/2
  Demux1/2 -> Mux/3
  Demux1/3 -> Mux/4
  Demux/1 -> Mux/6
  Demux/2 -> Mux/7
  Demux1/1 -> Mux/8
  Mux/1 -> Reshape/1
  Reshape/1 -> Product/1
  B/1 -> Product/2

== system gtm_design/GTM_T2/Engines/Left_Engine Jetcat P70/Throttle Lag ==
  throttle : Inport
  Gain : Gain  Gain=B  Multiplication=Matrix(K*u)
  Gain1 : Gain  Gain=A  Multiplication=Matrix(K*u)
  Gain2 : Gain  Gain=C  Multiplication=Matrix(K*u)
  Gain3 : Gain  Gain=flipud(B)/C(2)
  Integrator : Integrator  InitialConditionSource=external
  Sum1 : Sum  Inputs=|++
  y : Outport  VectorParamsAs1DForOutWhenUnconnected=off
  wires:
  Gain3/1 -> Integrator/2
  throttle/1 -> Gain3/1, Gain/1
  Gain2/1 -> y/1
  Gain/1 -> Sum1/1
  Integrator/1 -> Gain2/1, Gain1/1
  Gain1/1 -> Sum1/2
  Sum1/1 -> Integrator/1  "xdot"

== system gtm_design/GTM_T2/Engines/Right_Engine Jetcat P70/Throttle Lag ==
  throttle : Inport
  Gain : Gain  Gain=B  Multiplication=Matrix(K*u)
  Gain1 : Gain  Gain=A  Multiplication=Matrix(K*u)
  Gain2 : Gain  Gain=C  Multiplication=Matrix(K*u)
  Gain3 : Gain  Gain=flipud(B)/C(2)
  Integrator : Integrator  InitialConditionSource=external
  Sum1 : Sum  Inputs=|++
  y : Outport  VectorParamsAs1DForOutWhenUnconnected=off
  wires:
  Gain3/1 -> Integrator/2
  throttle/1 -> Gain3/1, Gain/1
  Gain2/1 -> y/1
  Gain/1 -> Sum1/1
  Integrator/1 -> Gain2/1, Gain1/1
  Gain1/1 -> Sum1/2
  Sum1/1 -> Integrator/1  "xdot"

== system gtm_design/GTM_T2/Landing Gear/LandingGear/Euler to DCM1 ==
  "Euler " : Inport
  Fcn : Fcn  Expr=u(4)*u(2)*u(6)+u(3)*u(1)
  Fcn1 : Fcn  Expr=u(3)*u(5)
  Fcn2 : Fcn  Expr=u(3)*u(2)*u(1)+u(6)*u(4)
  Fcn3 : Fcn  Expr=u(3)*u(2)*u(4)-u(6)*u(1)
  Fcn4 : Fcn  Expr=-u(2)
  Fcn5 : Fcn  Expr=u(5)*u(1)
  Fcn6 : Fcn  Expr=u(1)*u(2)*u(6)-u(3)*u(4)
  Fcn7 : Fcn  Expr=u(5)*u(6)
  Fcn8 : Fcn  Expr=u(5)*u(4)
  Mux : Mux  Inputs=2
  Mux1 : Mux  Inputs=9
  Reshape : Reshape  OutputDimensionality=Customize  OutputDimensions=[3,3]
  Trigonometric Function : Trigonometry
  Trigonometric Function1 : Trigonometry  Operator=cos
  DCM : Outport  VectorParamsAs1DForOutWhenUnconnected=off
  wires:
  "Euler "/1 -> Trigonometric Function1/1, Trigonometric Function/1
  Trigonometric Function/1 -> Mux/1
  Trigonometric Function1/1 -> Mux/2
  Mux/1 -> Fcn/1, Fcn7/1, Fcn6/1, Fcn1/1, Fcn2/1, Fcn4/1, Fcn8/1, Fcn5/1, Fcn3/1
  Mux1/1 -> Reshape/1
  Fcn7/1 -> Mux1/1
  Fcn6/1 -> Mux1/2
  Fcn/1 -> Mux1/3
  Fcn1/1 -> Mux1/4
  Fcn2/1 -> Mux1/5
  Fcn3/1 -> Mux1/6
  Fcn4/1 -> Mux1/7
  Fcn5/1 -> Mux1/8
  Fcn8/1 -> Mux1/9
  Reshape/1 -> DCM/1

== system gtm_design/GTM_T2/Landing Gear/LandingGear/Subsystem ==
  Alt : Inport
  Mux : Mux  Inputs=2
  Sum : Sum  Inputs=|+-
  Wheel Positions3 : Constant  Value=RunwayAlt
  Wheel Positions4 : Constant  Value=[0;0]
  cg_wrt_rwy : Outport  VectorParamsAs1DForOutWhenUnconnected=off
  wires:
  Mux/1 -> cg_wrt_rwy/1
  Sum/1 -> Mux/2
  Alt/1 -> Sum/1
  Wheel Positions4/1 -> Mux/1
  Wheel Positions3/1 -> Sum/2

== system gtm_design/GTM_T2/Sensors/Air Data/First Order Filter ==
  In : Inport
  Constant : Constant  Value=Timestep
  Constant1 : Constant  Value=tau
  Enabled Subsystem : Subsystem  TreatAsAtomicUnit=on
  Relational Operator : RelationalOperator  Operator=>  OutDataTypeStr=boolean  RndMeth=Nearest
  Switch : Switch  Threshold=0.5
  Out : Outport  VectorParamsAs1DForOutWhenUnconnected=off
  wires:
  Constant1/1 -> Enabled Subsystem/2(tau), Relational Operator/1
  Enabled Subsystem/1(Out) -> Switch/1
  Switch/1 -> Out/1
  In/1 -> Enabled Subsystem/1(In), Switch/3
  Relational Operator/1 -> Enabled Subsystem/Enable, Switch/2
  Constant/1 -> Relational Operator/2

== system gtm_design/GTM_T2/Sensors/Air Data/Sensor Model1 ==
  In1 : Inport
  Add : Sum  Inputs=+++
  Gain : Gain  Gain=scf
  Gear1 : Constant  Value=bias
  Gear2 : Constant  Value=noise_on
  Noise_on : Switch  Threshold=0.5  SaturateOnIntegerOverflow=on  InputSameDT=on
  White Noise : RandomNumber  Variance=sigma*sigma  Seed=round(seed*rand(1))  SampleTime=Timestep
  Out1 : Outport  VectorParamsAs1DForOutWhenUnconnected=off
  wires:
  Noise_on/1 -> Out1/1
  Gear2/1 -> Noise_on/2
  White Noise/1 -> Add/1
  Add/1 -> Noise_on/1
  Gear1/1 -> Add/2
  Gain/1 -> Add/3
  In1/1 -> Noise_on/3, Gain/1

== system gtm_design/GTM_T2/Sensors/Air Data/Sensor Model2 ==
  In1 : Inport
  Add : Sum  Inputs=+++
  Gain : Gain  Gain=scf
  Gear1 : Constant  Value=bias
  Gear2 : Constant  Value=noise_on
  Noise_on : Switch  Threshold=0.5  SaturateOnIntegerOverflow=on  InputSameDT=on
  White Noise : RandomNumber  Variance=sigma*sigma  Seed=round(seed*rand(1))  SampleTime=Timestep
  Out1 : Outport  VectorParamsAs1DForOutWhenUnconnected=off
  wires:
  Noise_on/1 -> Out1/1
  Gear2/1 -> Noise_on/2
  White Noise/1 -> Add/1
  Add/1 -> Noise_on/1
  Gear1/1 -> Add/2
  Gain/1 -> Add/3
  In1/1 -> Noise_on/3, Gain/1

== system gtm_design/GTM_T2/Sensors/Air Data/Sensor Model3 ==
  In1 : Inport
  Add : Sum  Inputs=+++
  Gain : Gain  Gain=scf
  Gear1 : Constant  Value=bias
  Gear2 : Constant  Value=noise_on
  Noise_on : Switch  Threshold=0.5  SaturateOnIntegerOverflow=on  InputSameDT=on
  White Noise : RandomNumber  Variance=sigma*sigma  Seed=round(seed*rand(1))  SampleTime=Timestep
  Out1 : Outport  VectorParamsAs1DForOutWhenUnconnected=off
  wires:
  Noise_on/1 -> Out1/1
  Gear2/1 -> Noise_on/2
  White Noise/1 -> Add/1
  Add/1 -> Noise_on/1
  Gear1/1 -> Add/2
  Gain/1 -> Add/3
  In1/1 -> Noise_on/3, Gain/1

== system gtm_design/GTM_T2/Sensors/Air Data/Sensor Model4 ==
  In1 : Inport
  Add : Sum  Inputs=+++
  Gain : Gain  Gain=scf
  Gear1 : Constant  Value=bias
  Gear2 : Constant  Value=noise_on
  Noise_on : Switch  Threshold=0.5  SaturateOnIntegerOverflow=on  InputSameDT=on
  White Noise : RandomNumber  Variance=sigma*sigma  Seed=round(seed*rand(1))  SampleTime=Timestep
  Out1 : Outport  VectorParamsAs1DForOutWhenUnconnected=off
  wires:
  Noise_on/1 -> Out1/1
  Gear2/1 -> Noise_on/2
  White Noise/1 -> Add/1
  Add/1 -> Noise_on/1
  Gear1/1 -> Add/2
  Gain/1 -> Add/3
  In1/1 -> Noise_on/3, Gain/1

== system gtm_design/GTM_T2/Sensors/Air Data/Sensor Model5 ==
  In1 : Inport
  Add : Sum  Inputs=+++
  Gain : Gain  Gain=scf
  Gear1 : Constant  Value=bias
  Gear2 : Constant  Value=noise_on
  Noise_on : Switch  Threshold=0.5  SaturateOnIntegerOverflow=on  InputSameDT=on
  White Noise : RandomNumber  Variance=sigma*sigma  Seed=round(seed*rand(1))  SampleTime=Timestep
  Out1 : Outport  VectorParamsAs1DForOutWhenUnconnected=off
  wires:
  Noise_on/1 -> Out1/1
  Gear2/1 -> Noise_on/2
  White Noise/1 -> Add/1
  Add/1 -> Noise_on/1
  Gear1/1 -> Add/2
  Gain/1 -> Add/3
  In1/1 -> Noise_on/3, Gain/1

== system gtm_design/GTM_T2/Sensors/Air Data/Sensor Model6 ==
  In1 : Inport
  Add : Sum  Inputs=+++
  Gain : Gain  Gain=scf
  Gear1 : Constant  Value=bias
  Gear2 : Constant  Value=noise_on
  Noise_on : Switch  Threshold=0.5  SaturateOnIntegerOverflow=on  InputSameDT=on
  White Noise : RandomNumber  Variance=sigma*sigma  Seed=round(seed*rand(1))  SampleTime=Timestep
  Out1 : Outport  VectorParamsAs1DForOutWhenUnconnected=off
  wires:
  Noise_on/1 -> Out1/1
  Gear2/1 -> Noise_on/2
  White Noise/1 -> Add/1
  Add/1 -> Noise_on/1
  Gear1/1 -> Add/2
  Gain/1 -> Add/3
  In1/1 -> Noise_on/3, Gain/1

== system gtm_design/GTM_T2/Sensors/MAG3 IMU/Sensor Model1 ==
  In1 : Inport
  Add : Sum  Inputs=+++
  Gain : Gain  Gain=scf
  Gear1 : Constant  Value=bias
  Gear2 : Constant  Value=noise_on
  Noise_on : Switch  Threshold=0.5  SaturateOnIntegerOverflow=on  InputSameDT=on
  White Noise : RandomNumber  Variance=sigma*sigma  Seed=round(seed*rand(1))  SampleTime=Timestep
  Out1 : Outport  VectorParamsAs1DForOutWhenUnconnected=off
  wires:
  Noise_on/1 -> Out1/1
  Gear2/1 -> Noise_on/2
  White Noise/1 -> Add/1
  Add/1 -> Noise_on/1
  Gear1/1 -> Add/2
  Gain/1 -> Add/3
  In1/1 -> Noise_on/3, Gain/1

== system gtm_design/GTM_T2/Sensors/MAG3 IMU/Sensor Model2 ==
  In1 : Inport
  Add : Sum  Inputs=+++
  Gain : Gain  Gain=scf
  Gear1 : Constant  Value=bias
  Gear2 : Constant  Value=noise_on
  Noise_on : Switch  Threshold=0.5  SaturateOnIntegerOverflow=on  InputSameDT=on
  White Noise : RandomNumber  Variance=sigma*sigma  Seed=round(seed*rand(1))  SampleTime=Timestep
  Out1 : Outport  VectorParamsAs1DForOutWhenUnconnected=off
  wires:
  Noise_on/1 -> Out1/1
  Gear2/1 -> Noise_on/2
  White Noise/1 -> Add/1
  Add/1 -> Noise_on/1
  Gear1/1 -> Add/2
  Gain/1 -> Add/3
  In1/1 -> Noise_on/3, Gain/1

== system gtm_design/GTM_T2/Sensors/MAG3 IMU/Sensor Model3 ==
  In1 : Inport
  Add : Sum  Inputs=+++
  Gain : Gain  Gain=scf
  Gear1 : Constant  Value=bias
  Gear2 : Constant  Value=noise_on
  Noise_on : Switch  Threshold=0.5  SaturateOnIntegerOverflow=on  InputSameDT=on
  White Noise : RandomNumber  Variance=sigma*sigma  Seed=round(seed*rand(1))  SampleTime=Timestep
  Out1 : Outport  VectorParamsAs1DForOutWhenUnconnected=off
  wires:
  Noise_on/1 -> Out1/1
  Gear2/1 -> Noise_on/2
  White Noise/1 -> Add/1
  Add/1 -> Noise_on/1
  Gear1/1 -> Add/2
  Gain/1 -> Add/3
  In1/1 -> Noise_on/3, Gain/1

== system gtm_design/GTM_T2/Sensors/MAG3 IMU/Sensor Model4 ==
  In1 : Inport
  Add : Sum  Inputs=+++
  Gain : Gain  Gain=scf
  Gear1 : Constant  Value=bias
  Gear2 : Constant  Value=noise_on
  Noise_on : Switch  Threshold=0.5  SaturateOnIntegerOverflow=on  InputSameDT=on
  White Noise : RandomNumber  Variance=sigma*sigma  Seed=round(seed*rand(1))  SampleTime=Timestep
  Out1 : Outport  VectorParamsAs1DForOutWhenUnconnected=off
  wires:
  Noise_on/1 -> Out1/1
  Gear2/1 -> Noise_on/2
  White Noise/1 -> Add/1
  Add/1 -> Noise_on/1
  Gear1/1 -> Add/2
  Gain/1 -> Add/3
  In1/1 -> Noise_on/3, Gain/1

== system gtm_design/GTM_T2/Sensors/MAG3 IMU/Sensor Model5 ==
  In1 : Inport
  Add : Sum  Inputs=+++
  Gain : Gain  Gain=scf
  Gear1 : Constant  Value=bias
  Gear2 : Constant  Value=noise_on
  Noise_on : Switch  Threshold=0.5  SaturateOnIntegerOverflow=on  InputSameDT=on
  White Noise : RandomNumber  Variance=sigma*sigma  Seed=round(seed*rand(1))  SampleTime=Timestep
  Out1 : Outport  VectorParamsAs1DForOutWhenUnconnected=off
  wires:
  Noise_on/1 -> Out1/1
  Gear2/1 -> Noise_on/2
  White Noise/1 -> Add/1
  Add/1 -> Noise_on/1
  Gear1/1 -> Add/2
  Gain/1 -> Add/3
  In1/1 -> Noise_on/3, Gain/1

== system gtm_design/GTM_T2/Sensors/MAG3 IMU/Sensor Model6 ==
  In1 : Inport
  Add : Sum  Inputs=+++
  Gain : Gain  Gain=scf
  Gear1 : Constant  Value=bias
  Gear2 : Constant  Value=noise_on
  Noise_on : Switch  Threshold=0.5  SaturateOnIntegerOverflow=on  InputSameDT=on
  White Noise : RandomNumber  Variance=sigma*sigma  Seed=round(seed*rand(1))  SampleTime=Timestep
  Out1 : Outport  VectorParamsAs1DForOutWhenUnconnected=off
  wires:
  Noise_on/1 -> Out1/1
  Gear2/1 -> Noise_on/2
  White Noise/1 -> Add/1
  Add/1 -> Noise_on/1
  Gear1/1 -> Add/2
  Gain/1 -> Add/3
  In1/1 -> Noise_on/3, Gain/1
